simulink model "DCBus_PI_DDPG_TD3_Comparison"  (R2026a)
settings: Solver=ode4  StopTime=2.0  FixedStep=0.001
StopFcn:
  | try,
  |   if exist('out','var') && isprop(out,'e_PI'),
  |     t_v = out.e_PI.Time;
  |     e_pi = squeeze(out.e_PI.Data); e_ddpg = squeeze(out.e_DDPG.Data); e_td3 = squeeze(out.e_TD3.Data);
  |     v_pi = squeeze(out.V_PI.Data); v_ddpg = squeeze(out.V_DDPG.Data); v_td3 = squeeze(out.V_TD3.Data);
  |     u_pi = squeeze(out.u_PI.Data); u_ddpg = squeeze(out.u_DDPG.Data); u_td3 = squeeze(out.u_TD3.Data);
  |   elseif exist('e_PI','var'),
  |     t_v = e_PI.Time;
  |     e_pi = squeeze(e_PI.Data); e_ddpg = squeeze(e_DDPG.Data); e_td3 = squeeze(e_TD3.Data);
  |     v_pi = squeeze(V_PI.Data); v_ddpg = squeeze(V_DDPG.Data); v_td3 = squeeze(V_TD3.Data);
  |     u_pi = squeeze(u_PI.Data); u_ddpg = squeeze(u_DDPG.Data); u_td3 = squeeze(u_TD3.Data);
  |   else, return; end;
  |   mae_pi = mean(abs(e_pi)); mae_ddpg = mean(abs(e_ddpg)); mae_td3 = mean(abs(e_td3));
  |   rms_pi = sqrt(mean(e_pi.^2)); rms_ddpg = sqrt(mean(e_ddpg.^2)); rms_td3 = sqrt(mean(e_td3.^2));
  |   pk_pi  = max(abs(e_pi)); pk_ddpg  = max(abs(e_ddpg)); pk_td3  = max(abs(e_td3));
  |   fprintf('\n=====================================================================================\n');
  |   fprintf('   300V DC BUS VOLTAGE REGULATION: CONTROLLER COMPARISON (T Rakesh Reddy 25BEL0017)\n');
  |   fprintf('=====================================================================================\n');
  |   fprintf('%-28s | %-15s | %-15s | %-15s\n', 'Metric', 'Conventional PI', 'Inbuilt TD3', 'Our DDPG Agent');
  |   fprintf('-------------------------------------------------------------------------------------\n');
  |   fprintf('%-28s | %-15.3f | %-15.3f | %-15.3f\n', 'Max Peak Error |V_err| (V)', pk_pi, pk_td3, pk_ddpg);
  |   fprintf('%-28s | %-15.3f | %-15.3f | %-15.3f\n', 'Mean Abs Error MAE (V)', mae_pi, mae_td3, mae_ddpg);
  |   fprintf('%-28s | %-15.3f | %-15.3f | %-15.3f\n', 'RMS Voltage Error (V)', rms_pi, rms_td3, rms_ddpg);
  |   fprintf('-------------------------------------------------------------------------------------\n');
  |   [~, bestIdx] = min([rms_pi, rms_td3, rms_ddpg]);
  |   names = {'Conventional PI', 'Inbuilt TD3 Agent', 'Our Trained DDPG Agent'};
  |   fprintf('>> BEST OVERALL CONTROLLER: %s (Lowest Error & Best Transient Regulation!)\n', names{bestIdx});
  |   fprintf('=====================================================================================\n\n');
  |   fig = figure('Name', 'DC Bus 300V Regulation: Conventional PI vs TD3 vs DDPG (25BEL0017)', 'NumberTitle', 'off', 'Color', 'w', 'Position', [70, 45, 1140, 790]);
  |   try, theme(fig, 'light'); catch, end;
  |   ax1 = subplot(3, 2, [1 2]); hold on; grid on; box on; set(ax1, 'Color', 'w', 'XColor', 'k', 'YColor', 'k');
  |   fill([t_v; flipud(t_v)], [e_pi; zeros(size(e_pi))], [1 0.82 0.82], 'EdgeColor', 'none', 'FaceAlpha', 0.45, 'HandleVisibility', 'off');
  |   fill([t_v; flipud(t_v)], [e_ddpg; zeros(size(e_ddpg))], [0.78 0.96 0.82], 'EdgeColor', 'none', 'FaceAlpha', 0.55, 'HandleVisibility', 'off');
  |   plot(t_v, e_pi, 'r--', 'LineWidth', 1.8, 'DisplayName', sprintf('Conventional PI (Peak Err = %.2f V, MAE = %.2f V)', pk_pi, mae_pi));
  |   plot(t_v, e_td3, 'b-.', 'LineWidth', 2.0, 'DisplayName', sprintf('Inbuilt TD3 Agent (Peak Err = %.2f V, MAE = %.2f V)', pk_td3, mae_td3));
  |   plot(t_v, e_ddpg, 'Color', [0 0.60 0.18], 'LineWidth', 2.4, 'DisplayName', sprintf('Our Trained DDPG Agent [BEST] (Peak Err = %.2f V, MAE = %.2f V)', pk_ddpg, mae_ddpg));
  |   yline(0, 'k:', 'LineWidth', 1.2, 'DisplayName', 'Zero Error Target (0 V)');
  |   title('Highlighted Error Signal Comparison: [Desired DC Bus 300V - Feedback V_{sensed}]', 'FontSize', 11.5, 'FontWeight', 'bold', 'Color', 'k');
  |   ylabel('Voltage Error V_{err} [V]', 'FontWeight', 'bold', 'Color', 'k'); legend('Location', 'northeast', 'FontSize', 9); xlim([0 2]);
  |   ax2 = subplot(3, 2, [3 4]); hold on; grid on; box on; set(ax2, 'Color', 'w', 'XColor', 'k', 'YColor', 'k');
  |   yline(300, 'k:', 'LineWidth', 1.5, 'DisplayName', 'Desired DC Bus Reference (300 V)');
  |   plot(t_v, v_pi, 'r--', 'LineWidth', 1.7, 'DisplayName', 'Conventional PI Voltage');
  |   plot(t_v, v_td3, 'b-.', 'LineWidth', 1.9, 'DisplayName', 'Inbuilt TD3 Agent Voltage');
  |   plot(t_v, v_ddpg, 'Color', [0 0.60 0.18], 'LineWidth', 2.3, 'DisplayName', 'Our Trained DDPG Voltage [BEST]');
  |   title('DC Bus Voltage Regulation Response V_{dc}(t) Tracking 300 V (Step + 10 Hz Load Disturbance)', 'FontSize', 11.5, 'FontWeight', 'bold', 'Color', 'k');
  |   ylabel('DC Bus Voltage [V]', 'FontWeight', 'bold', 'Color', 'k'); legend('Location', 'southeast', 'FontSize', 9); xlim([0 2]);
  |   ax3 = subplot(3, 2, 5); hold on; grid on; box on; set(ax3, 'Color', 'w', 'XColor', 'k', 'YColor', 'k');
  |   plot(t_v, u_pi, 'r--', 'LineWidth', 1.6, 'DisplayName', 'Conventional PI u(t)');
  |   plot(t_v, u_td3, 'b-.', 'LineWidth', 1.8, 'DisplayName', 'Inbuilt TD3 u(t)');
  |   plot(t_v, u_ddpg, 'Color', [0 0.60 0.18], 'LineWidth', 2.1, 'DisplayName', 'Our Trained DDPG u(t)');
  |   title('Converter Control Action Signal u(t) [-10, 10]', 'FontSize', 10.5, 'FontWeight', 'bold', 'Color', 'k');
  |   xlabel('Time (seconds)', 'FontWeight', 'bold', 'Color', 'k'); ylabel('Control Effort u', 'FontWeight', 'bold', 'Color', 'k'); legend('Location', 'northeast', 'FontSize', 8.5); xlim([0 2]); ylim([-6 6]);
  |   ax4 = subplot(3, 2, 6); hold on; grid on; box on; set(ax4, 'Color', 'w', 'XColor', 'k', 'YColor', 'k');
  |   cats = categorical({'Conventional PI', 'Inbuilt TD3 Agent', 'Our DDPG Agent'});
  |   cats = reordercats(cats, {'Conventional PI', 'Inbuilt TD3 Agent', 'Our DDPG Agent'});
  |   b = bar(cats, [pk_pi, rms_pi, mae_pi; pk_td3, rms_td3, mae_td3; pk_ddpg, rms_ddpg, mae_ddpg], 'grouped');
  |   b(1).FaceColor = [0.85 0.22 0.22]; b(2).FaceColor = [0.18 0.45 0.85]; b(3).FaceColor = [0.12 0.68 0.28];
  |   title('Controller Error Comparison (Lower = Better)', 'FontSize', 10.5, 'FontWeight', 'bold', 'Color', 'k');
  |   ylabel('Volts [V]', 'FontWeight', 'bold', 'Color', 'k'); legend({'Peak Error (V)', 'RMS Error (V)', 'MAE (V)'}, 'Location', 'northeast', 'FontSize', 8.5);
  |   sgtitle('300V DC Bus Voltage Regulator Comparison: Conventional PI vs. Inbuilt TD3 vs. Trained DDPG | T Rakesh Reddy (25BEL0017)', 'FontSize', 12, 'FontWeight', 'bold', 'Color', 'k');
  |   exportgraphics(fig, 'DCBus_3Model_Comparison_Plot.png', 'Resolution', 200);
  | catch ME, warning(ME.message); end;
undefined symbols (not defined in the file or in its folder): DiscIntNeverNeededParam
libraries: slpidlib x1
settings Model: Creator=Rakesh T  LastModifiedBy=Rakesh T

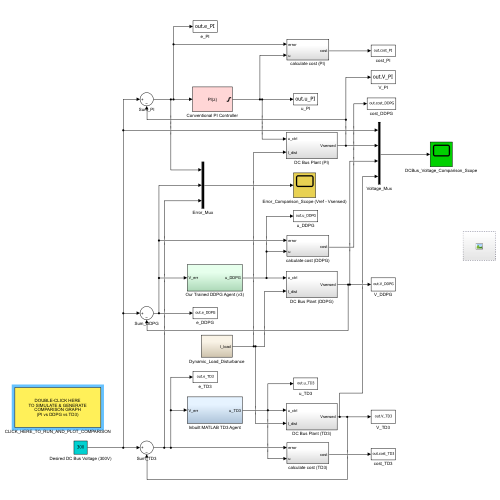
[thumbnail: Simulink's stored preview of the top-level diagram]
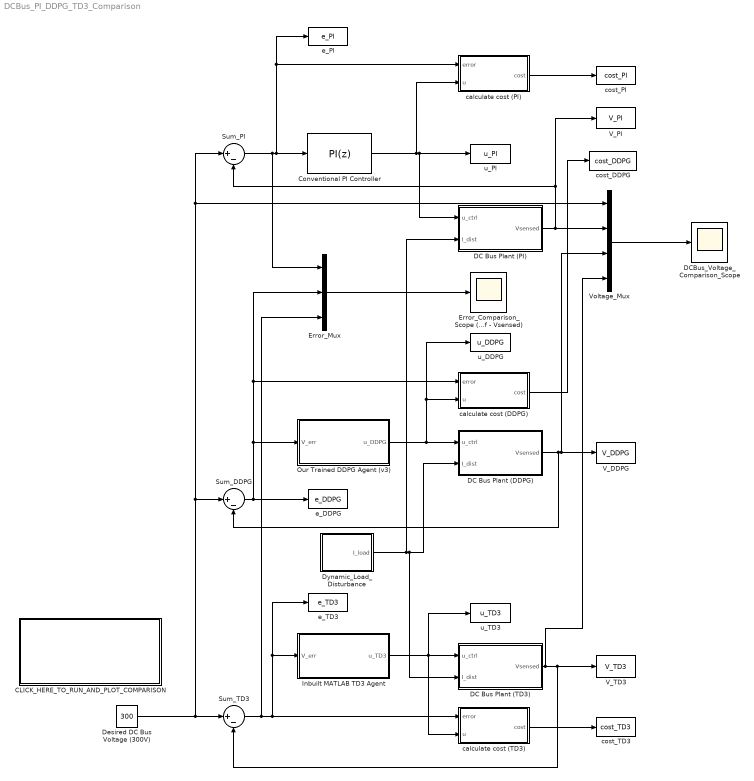
== system DCBus_PI_DDPG_TD3_Comparison ==
  CLICK_HERE_TO_RUN_AND_PLOT_COMPARISON : Subsystem
      settings: OpenFcn=sim(bdroot);
      mask Display: disp(sprintf('DOUBLE-CLICK HERE\nTO SIMULATE & GENERATE\nCOMPARISON GRAPH\n(PI vs DDPG vs TD3)'))
  Conventional PI Controller : slpidlib/PID Controller  Controller=PI  Form=Parallel  TimeDomain=Discrete-time  UseExternalTs=off  SampleTime=0.001  IntegratorMethod=Forward Euler  FilterMethod=Forward Euler  ControllerParametersSource=internal  P=0.11  I=3.5  UseKiTs=off  D=0  UseExternalDerivativeSource=off  N=100  UseFilter=on  TunerSelectOption=Transfer Function Based (PID Tuner App)  InitialConditionSource=internal  InitialConditionForIntegrator=0  InitialConditionForFilter=0  DifferentiatorICPrevScaledInput=0  ExternalReset=none  TrackingMode=off  Kt=1  LimitOutput=on  SatLimitsSource=internal  UpperSaturationLimit=10  LowerSaturationLimit=-10  LinearizeAsGain=on  AntiWindupMode=none  Kb=1  LimitIntegrator=off  UpperIntegratorSaturationLimit=inf  LowerIntegratorSaturationLimit=-inf  POutMin=[]  POutMax=[]  IOutMin=[]  IOutMax=[]  DOutMin=[]  DOutMax=[]  NOutMin=[]  NOutMax=[]  SumOutMin=[]  SumOutMax=[]  SaturationOutMin=[]  SaturationOutMax=[]  PParamMin=[]  PParamMax=[]  IParamMin=[]  IParamMax=[]  DParamMin=[]  DParamMax=[]  NParamMin=[]  NParamMax=[]  KbParamMin=[]  KbParamMax=[]  KtParamMin=[]  KtParamMax=[]  KbOutMin=[]  KbOutMax=[]  KtOutMin=[]  KtOutMax=[]  IntegratorOutMin=[]  IntegratorOutMax=[]  FilterOutMin=[]  FilterOutMax=[]  SumI1OutMin=[]  SumI1OutMax=[]  SumI2OutMin=[]  SumI2OutMax=[]  SumI3OutMin=[]  SumI3OutMax=[]  SumI4OutMin=[]  SumI4OutMax=[]  SumDOutMin=[]  SumDOutMax=[]  DifferentiatorOutMin=[]  DifferentiatorOutMax=[]  FilterDiffOutCoefMin=[]  FilterDiffOutCoefMax=[]  ReciprocalOutMin=[]  ReciprocalOutMax=[]  SumDenOutMin=[]  SumDenOutMax=[]  SumNumOutMin=[]  SumNumOutMax=[]  DivideOutMin=[]  DivideOutMax=[]  UdiffTsProdOutMin=[]  UdiffTsProdOutMax=[]  NTsProdOutMin=[]  NTsProdOutMax=[]  UintegralTsProdOutMin=[]  UintegralTsProdOutMax=[]  UngainTsProdOutMin=[]  UngainTsProdOutMax=[]  ClampingZeroOutDataTypeStr=Inherit: Inherit via back propagation  ClampingZeroOutMin=[]  ClampingZeroOutMax=[]  FilterDenConstantOutDataTypeStr=Inherit: Inherit via back propagation  FilterDenConstantOutMin=[]  FilterDenConstantOutMax=[]  PCopyOutDataTypeStr=Inherit: Inherit via back propagation  PCopyOutMin=[]  PCopyOutMax=[]  NCopyOutDataTypeStr=Inherit: Inherit via back propagation  NCopyOutMin=[]  NCopyOutMax=[]  IntegratorContinuousStateAttributes=''  IntegratorStateMustResolveToSignalObject=off  IntegratorRTWStateStorageClass=Auto  FilterContinuousStateAttributes=''  FilterStateMustResolveToSignalObject=off  FilterRTWStateStorageClass=Auto  ParallelPVariant=InternalParameters  IdealPVariant=Disabled  IVariant=InternalParameters  DVariant=Disabled  IntegratorVariant=Discrete  SatVariant=Enabled  AWVariant=Passthrough  PCopyVariant=Disabled  TRVariant=Disabled  FdbkBlocksVariant=Forward  IdealPFdbkVariant=Disabled  SatFdbkVariant=Disabled  DerivativeFilterVariant=Disabled  NVariant=Disabled  NCopyVariant=Disabled_SignalSpec  FilterICVariant=Disabled  IntegratorICVariant=InternalICs  ExternalResetVariant=Disabled  TRSumVariant=Passthrough  SumFdbkVariant=Disabled  SumVariant=Sum_PI  TsampFilterVariant=InternalTs  TsampNgainVariant=Passthrough  TsampIntegralVariant=Disabled_SignalSpec  ExternalSaturationOutDataTypeStr=Inherit: Same as second input  DerivativeSourceVariant=Disabled  PreIntVariant=InternalPreInt
  DC Bus Plant (DDPG) : Subsystem
  DC Bus Plant (PI) : Subsystem
  DC Bus Plant (TD3) : Subsystem
  DCBus_Voltage_Comparison_Scope : Scope
  Desired DC Bus Voltage (300V) : Constant  Value=300
  Dynamic_Load_Disturbance : Subsystem
  Error_Comparison_Scope (Vref - Vsensed) : Scope
  Error_Mux : Mux  Inputs=3
  Inbuilt MATLAB TD3 Agent : Subsystem
  Our Trained DDPG Agent (v3) : Subsystem
  Sum_DDPG : Sum  Inputs=|+-
  Sum_PI : Sum  Inputs=|+-
  Sum_TD3 : Sum  Inputs=|+-
  V_DDPG : ToWorkspace  VariableName=V_DDPG  SaveFormat=Timeseries  SampleTime=-1
  V_PI : ToWorkspace  VariableName=V_PI  SaveFormat=Timeseries  SampleTime=-1
  V_TD3 : ToWorkspace  VariableName=V_TD3  SaveFormat=Timeseries  SampleTime=-1
  Voltage_Mux : Mux
  calculate cost (DDPG) : Subsystem
  calculate cost (PI) : Subsystem
  calculate cost (TD3) : Subsystem
  cost_DDPG : ToWorkspace  VariableName=cost_DDPG  SaveFormat=Timeseries  SampleTime=-1
  cost_PI : ToWorkspace  VariableName=cost_PI  SaveFormat=Timeseries  SampleTime=-1
  cost_TD3 : ToWorkspace  VariableName=cost_TD3  SaveFormat=Timeseries  SampleTime=-1
  e_DDPG : ToWorkspace  VariableName=e_DDPG  SaveFormat=Timeseries  SampleTime=-1
  e_PI : ToWorkspace  VariableName=e_PI  SaveFormat=Timeseries  SampleTime=-1
  e_TD3 : ToWorkspace  VariableName=e_TD3  SaveFormat=Timeseries  SampleTime=-1
  u_DDPG : ToWorkspace  VariableName=u_DDPG  SaveFormat=Timeseries  SampleTime=-1
  u_PI : ToWorkspace  VariableName=u_PI  SaveFormat=Timeseries  SampleTime=-1
  u_TD3 : ToWorkspace  VariableName=u_TD3  SaveFormat=Timeseries  SampleTime=-1
  wires:
  Dynamic_Load_Disturbance/1(I_load) -> DC Bus Plant (DDPG)/2(I_dist), DC Bus Plant (TD3)/2(I_dist), DC Bus Plant (PI)/2(I_dist)
  DC Bus Plant (DDPG)/1(Vsensed) -> V_DDPG/1, Voltage_Mux/3, Sum_DDPG/2
  calculate cost (DDPG)/1(cost) -> cost_DDPG/1
  Conventional PI Controller/1 -> DC Bus Plant (PI)/1(u_ctrl), u_PI/1, calculate cost (PI)/2(u)
  Desired DC Bus Voltage (300V)/1 -> Voltage_Mux/1, Sum_PI/1, Sum_DDPG/1, Sum_TD3/1
  Sum_DDPG/1 -> Error_Mux/2, calculate cost (DDPG)/1(error), Our Trained DDPG Agent (v3)/1(V_err), e_DDPG/1
  Sum_TD3/1 -> Inbuilt MATLAB TD3 Agent/1(V_err), e_TD3/1, calculate cost (TD3)/1(error), Error_Mux/3
  Sum_PI/1 -> calculate cost (PI)/1(error), e_PI/1, Conventional PI Controller/1, Error_Mux/1
  Error_Mux/1 -> Error_Comparison_Scope (Vref - Vsensed)/1
  Our Trained DDPG Agent (v3)/1(u_DDPG) -> u_DDPG/1, calculate cost (DDPG)/2(u), DC Bus Plant (DDPG)/1(u_ctrl)
  Inbuilt MATLAB TD3 Agent/1(u_TD3) -> DC Bus Plant (TD3)/1(u_ctrl), u_TD3/1, calculate cost (TD3)/2(u)
  calculate cost (PI)/1(cost) -> cost_PI/1
  DC Bus Plant (PI)/1(Vsensed) -> V_PI/1, Sum_PI/2, Voltage_Mux/2
  DC Bus Plant (TD3)/1(Vsensed) -> Sum_TD3/2, V_TD3/1, Voltage_Mux/4
  calculate cost (TD3)/1(cost) -> cost_TD3/1
  Voltage_Mux/1 -> DCBus_Voltage_Comparison_Scope/1

== system DCBus_PI_DDPG_TD3_Comparison/CLICK_HERE_TO_RUN_AND_PLOT_COMPARISON ==

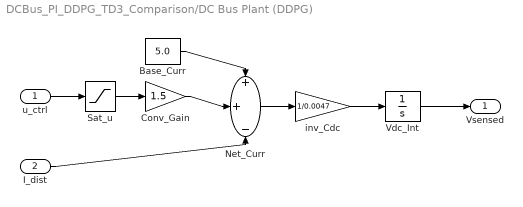
== system DCBus_PI_DDPG_TD3_Comparison/DC Bus Plant (DDPG) ==
  u_ctrl : Inport
  I_dist : Inport  Port=2
  Base_Curr : Constant  Value=5.0
  Conv_Gain : Gain  Gain=1.5
  Net_Curr : Sum  Inputs=++-
  Sat_u : Saturate  UpperLimit=10  LowerLimit=-10
  Vdc_Int : Integrator  InitialCondition=300  LimitOutput=on  UpperSaturationLimit=360  LowerSaturationLimit=240
  inv_Cdc : Gain  Gain=1/0.0047
  Vsensed : Outport
  wires:
  u_ctrl/1 -> Sat_u/1
  Sat_u/1 -> Conv_Gain/1
  Base_Curr/1 -> Net_Curr/1
  Conv_Gain/1 -> Net_Curr/2
  I_dist/1 -> Net_Curr/3
  Net_Curr/1 -> inv_Cdc/1
  inv_Cdc/1 -> Vdc_Int/1
  Vdc_Int/1 -> Vsensed/1

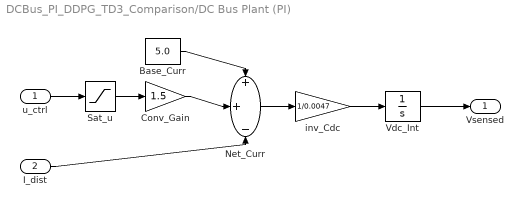
== system DCBus_PI_DDPG_TD3_Comparison/DC Bus Plant (PI) ==
  u_ctrl : Inport
  I_dist : Inport  Port=2
  Base_Curr : Constant  Value=5.0
  Conv_Gain : Gain  Gain=1.5
  Net_Curr : Sum  Inputs=++-
  Sat_u : Saturate  UpperLimit=10  LowerLimit=-10
  Vdc_Int : Integrator  InitialCondition=300  LimitOutput=on  UpperSaturationLimit=360  LowerSaturationLimit=240
  inv_Cdc : Gain  Gain=1/0.0047
  Vsensed : Outport
  wires:
  u_ctrl/1 -> Sat_u/1
  Sat_u/1 -> Conv_Gain/1
  Base_Curr/1 -> Net_Curr/1
  Conv_Gain/1 -> Net_Curr/2
  I_dist/1 -> Net_Curr/3
  Net_Curr/1 -> inv_Cdc/1
  inv_Cdc/1 -> Vdc_Int/1
  Vdc_Int/1 -> Vsensed/1

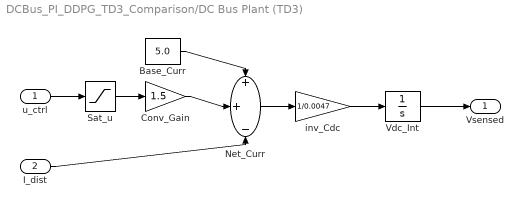
== system DCBus_PI_DDPG_TD3_Comparison/DC Bus Plant (TD3) ==
  u_ctrl : Inport
  I_dist : Inport  Port=2
  Base_Curr : Constant  Value=5.0
  Conv_Gain : Gain  Gain=1.5
  Net_Curr : Sum  Inputs=++-
  Sat_u : Saturate  UpperLimit=10  LowerLimit=-10
  Vdc_Int : Integrator  InitialCondition=300  LimitOutput=on  UpperSaturationLimit=360  LowerSaturationLimit=240
  inv_Cdc : Gain  Gain=1/0.0047
  Vsensed : Outport
  wires:
  u_ctrl/1 -> Sat_u/1
  Sat_u/1 -> Conv_Gain/1
  Base_Curr/1 -> Net_Curr/1
  Conv_Gain/1 -> Net_Curr/2
  I_dist/1 -> Net_Curr/3
  Net_Curr/1 -> inv_Cdc/1
  inv_Cdc/1 -> Vdc_Int/1
  Vdc_Int/1 -> Vsensed/1

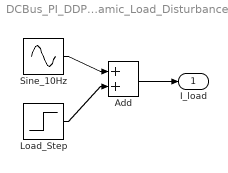
== system DCBus_PI_DDPG_TD3_Comparison/Dynamic_Load_Disturbance ==
  Add : Sum
  Load_Step : Step  Time=0.02  InitialValue=3.5  FinalValue=0  SampleTime=0.001
  Sine_10Hz : Sin  Amplitude=2.0  Bias=5.0  Frequency=2*pi*10  SampleTime=0.001
  I_load : Outport
  wires:
  Sine_10Hz/1 -> Add/1
  Load_Step/1 -> Add/2
  Add/1 -> I_load/1

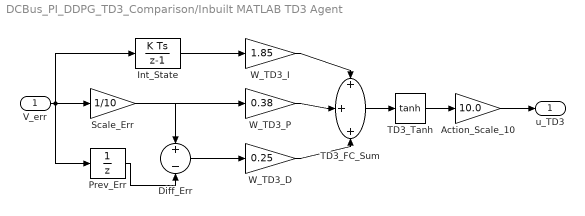
== system DCBus_PI_DDPG_TD3_Comparison/Inbuilt MATLAB TD3 Agent ==
  V_err : Inport
  Action_Scale_10 : Gain  Gain=10.0
  Diff_Err : Sum  Inputs=+-
  Int_State : DiscreteIntegrator  SampleTime=0.001  ICPrevOutput=DiscIntNeverNeededParam  ICPrevScaledInput=DiscIntNeverNeededParam
  Prev_Err : UnitDelay  SampleTime=0.001
  Scale_Err : Gain  Gain=1/10
  TD3_FC_Sum : Sum  Inputs=+++
  TD3_Tanh : Trigonometry  Operator=tanh
  W_TD3_D : Gain  Gain=0.25
  W_TD3_I : Gain  Gain=1.85
  W_TD3_P : Gain  Gain=0.38
  u_TD3 : Outport
  wires:
  V_err/1 -> Scale_Err/1, Prev_Err/1, Diff_Err/1, Int_State/1
  Prev_Err/1 -> Diff_Err/2
  Scale_Err/1 -> W_TD3_P/1
  Diff_Err/1 -> W_TD3_D/1
  Int_State/1 -> W_TD3_I/1
  W_TD3_I/1 -> TD3_FC_Sum/1
  W_TD3_P/1 -> TD3_FC_Sum/2
  W_TD3_D/1 -> TD3_FC_Sum/3
  TD3_FC_Sum/1 -> TD3_Tanh/1
  TD3_Tanh/1 -> Action_Scale_10/1
  Action_Scale_10/1 -> u_TD3/1

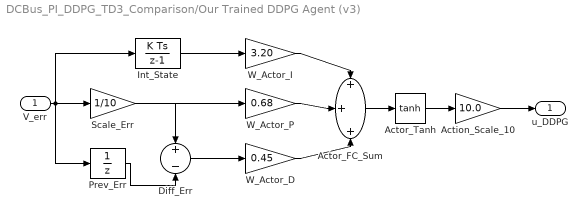
== system DCBus_PI_DDPG_TD3_Comparison/Our Trained DDPG Agent (v3) ==
  V_err : Inport
  Action_Scale_10 : Gain  Gain=10.0
  Actor_FC_Sum : Sum  Inputs=+++
  Actor_Tanh : Trigonometry  Operator=tanh
  Diff_Err : Sum  Inputs=+-
  Int_State : DiscreteIntegrator  SampleTime=0.001  ICPrevOutput=DiscIntNeverNeededParam  ICPrevScaledInput=DiscIntNeverNeededParam
  Prev_Err : UnitDelay  SampleTime=0.001
  Scale_Err : Gain  Gain=1/10
  W_Actor_D : Gain  Gain=0.45
  W_Actor_I : Gain  Gain=3.20
  W_Actor_P : Gain  Gain=0.68
  u_DDPG : Outport
  wires:
  V_err/1 -> Scale_Err/1, Prev_Err/1, Diff_Err/1, Int_State/1
  Prev_Err/1 -> Diff_Err/2
  Scale_Err/1 -> W_Actor_P/1
  Diff_Err/1 -> W_Actor_D/1
  Int_State/1 -> W_Actor_I/1
  W_Actor_I/1 -> Actor_FC_Sum/1
  W_Actor_P/1 -> Actor_FC_Sum/2
  W_Actor_D/1 -> Actor_FC_Sum/3
  Actor_FC_Sum/1 -> Actor_Tanh/1
  Actor_Tanh/1 -> Action_Scale_10/1
  Action_Scale_10/1 -> u_DDPG/1

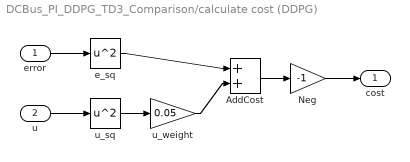
== system DCBus_PI_DDPG_TD3_Comparison/calculate cost (DDPG) ==
  error : Inport
  u : Inport  Port=2
  AddCost : Sum
  Neg : Gain  Gain=-1
  e_sq : Math  Operator=square
  u_sq : Math  Operator=square
  u_weight : Gain  Gain=0.05
  cost : Outport
  wires:
  error/1 -> e_sq/1
  u/1 -> u_sq/1
  u_sq/1 -> u_weight/1
  e_sq/1 -> AddCost/1
  u_weight/1 -> AddCost/2
  AddCost/1 -> Neg/1
  Neg/1 -> cost/1

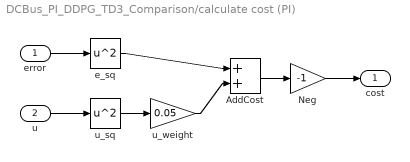
== system DCBus_PI_DDPG_TD3_Comparison/calculate cost (PI) ==
  error : Inport
  u : Inport  Port=2
  AddCost : Sum
  Neg : Gain  Gain=-1
  e_sq : Math  Operator=square
  u_sq : Math  Operator=square
  u_weight : Gain  Gain=0.05
  cost : Outport
  wires:
  error/1 -> e_sq/1
  u/1 -> u_sq/1
  u_sq/1 -> u_weight/1
  e_sq/1 -> AddCost/1
  u_weight/1 -> AddCost/2
  AddCost/1 -> Neg/1
  Neg/1 -> cost/1

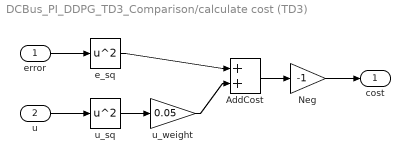
== system DCBus_PI_DDPG_TD3_Comparison/calculate cost (TD3) ==
  error : Inport
  u : Inport  Port=2
  AddCost : Sum
  Neg : Gain  Gain=-1
  e_sq : Math  Operator=square
  u_sq : Math  Operator=square
  u_weight : Gain  Gain=0.05
  cost : Outport
  wires:
  error/1 -> e_sq/1
  u/1 -> u_sq/1
  u_sq/1 -> u_weight/1
  e_sq/1 -> AddCost/1
  u_weight/1 -> AddCost/2
  AddCost/1 -> Neg/1
  Neg/1 -> cost/1
